simulink model "LQRconlacnguoc"  (R2024b)
settings: Solver=ode45  StartTime=0.0  StopTime=60  FixedStep=0.001  MaxStep=0.01  RelTol=1e-3
values from neighbouring files (symbols this model uses):
  D = [0; 0]    [K_vector_2.m]
libraries: simulink x20, slpidlib x11, slctrl_smc x5, mpclib x1, dspstat3 x1, rllib x1
(part 2 of 3)

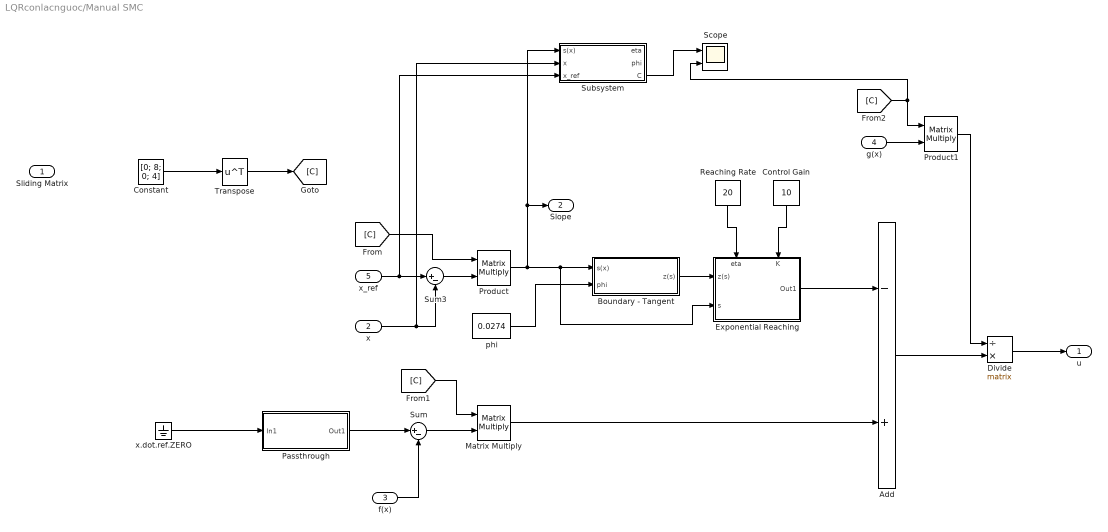
== system LQRconlacnguoc/Manual SMC ==
  Sliding Matrix : Inport
  x : Inport  Port=2
  f(x) : Inport  Port=3
  g(x) : Inport  Port=4
  x_ref : Inport  Port=5
  Add : Sum  Inputs=-+
  Boundary - Tangent : Subsystem
  Constant : Constant  Value=[0; 8; 0; 4]  VectorParams1D=off
  Control Gain : Constant  Value=10
  Divide : Product  Inputs=/*  Multiplication=Matrix(*)
  Exponential Reaching : Subsystem
      settings: PortSchema="{\"entries\":[{\"content\":{\"sides\":[{\"content\":{\"connectorIds\":[\"In1\",\"In2\"]},\"type\":\"ConnectorPlacement.EquallySpacedRectSide\",\"uuid\":\"14532932-ba42-4254-ad37-14ae2c40c086\"},{\"content\":{\"connectorIds\":[\"Out1\"],\"side\":\"RIGHT\"},\"type\":\"ConnectorPlacement.EquallySpacedRectSide\",\"uuid\":\"b67c1209-83dd-4fb0-99c8-05226babf43d\"},{\"content\":{\"connectorIds\":[\"In3\",\"In4\"],\"side\":\"TOP\"},\"type\":\"ConnectorPlacement.EquallySpacedRectSide\",\"uuid\":\"11cfd510-8790-4762-abc8-282610a147ed\"}]},\"type\":\"ConnectorPlacement.EquallySpacedConnector\",\"uuid\":\"c799e45e-6b6c-4526-9867-c33aadee095c\"}],\"packageUris\":[\"http://schema.mathworks.com/mf0/Connector/R2020b\"],\"version\":\"1.0\"}"
  Matrix Multiply : Product  Multiplication=Matrix(*)
  Passthrough : Subsystem  Variant=on
  Product : Product  Multiplication=Matrix(*)
  Product1 : Product  Multiplication=Matrix(*)
  Reaching Rate : Constant  Value=20
  Scope : Scope  NumInputPorts=2
  Subsystem : Subsystem
  Sum : Sum  Inputs=|+-
  Sum3 : Sum  Inputs=|+-
  Transpose : Math  Operator=transpose
  phi : Constant  Value=0.0274
  x.dot.ref.ZERO : Ground
  u : Outport
  Slope : Outport  Port=2
  wires:
  Transpose/1 -> [C]
  [C] -> Product/1
  x/1 -> Subsystem/2(x), Sum3/2
  x_ref/1 -> Subsystem/3(x_ref), Sum3/1
  Sum3/1 -> Product/2
  x.dot.ref.ZERO/1 -> Passthrough/1(In1)
  Passthrough/1(Out1) -> Sum/1
  f(x)/1 -> Sum/2
  Sum/1 -> Matrix Multiply/2
  [C] -> Matrix Multiply/1
  Product/1 -> Subsystem/1(s(x)), Slope/1, Exponential Reaching/2(s), Boundary - Tangent/1(s(x))
  phi/1 -> Boundary - Tangent/2(phi)
  Reaching Rate/1 -> Exponential Reaching/3(eta)
  Control Gain/1 -> Exponential Reaching/4(K)
  Boundary - Tangent/1(z(s)) -> Exponential Reaching/1(z(s))
  Exponential Reaching/1(Out1) -> Add/1
  Matrix Multiply/1 -> Add/2
  [C] -> Scope/2, Product1/1
  g(x)/1 -> Product1/2
  Add/1 -> Divide/2
  Product1/1 -> Divide/1
  Divide/1 -> u/1
  Constant/1 -> Transpose/1
  Subsystem/3(C) -> Scope/1

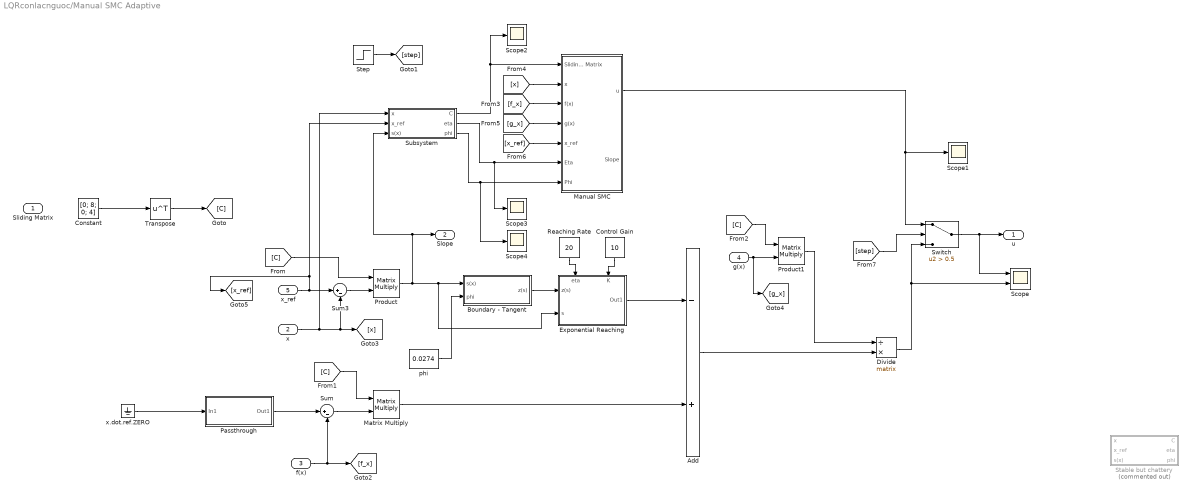
== system LQRconlacnguoc/Manual SMC Adaptive ==
  Sliding Matrix : Inport
  x : Inport  Port=2
  f(x) : Inport  Port=3
  g(x) : Inport  Port=4
  x_ref : Inport  Port=5
  Add : Sum  Inputs=-+
  Boundary - Tangent : Subsystem
  Constant : Constant  Value=[0; 8; 0; 4]  VectorParams1D=off
  Control Gain : Constant  Value=10
  Divide : Product  Inputs=/*  Multiplication=Matrix(*)
  Exponential Reaching : Subsystem
      settings: PortSchema="{\"entries\":[{\"content\":{\"sides\":[{\"content\":{\"connectorIds\":[\"In1\",\"In2\"]},\"type\":\"ConnectorPlacement.EquallySpacedRectSide\",\"uuid\":\"14532932-ba42-4254-ad37-14ae2c40c086\"},{\"content\":{\"connectorIds\":[\"Out1\"],\"side\":\"RIGHT\"},\"type\":\"ConnectorPlacement.EquallySpacedRectSide\",\"uuid\":\"b67c1209-83dd-4fb0-99c8-05226babf43d\"},{\"content\":{\"connectorIds\":[\"In3\",\"In4\"],\"side\":\"TOP\"},\"type\":\"ConnectorPlacement.EquallySpacedRectSide\",\"uuid\":\"11cfd510-8790-4762-abc8-282610a147ed\"}]},\"type\":\"ConnectorPlacement.EquallySpacedConnector\",\"uuid\":\"c799e45e-6b6c-4526-9867-c33aadee095c\"}],\"packageUris\":[\"http://schema.mathworks.com/mf0/Connector/R2020b\"],\"version\":\"1.0\"}"
  Manual SMC : Subsystem
  Matrix Multiply : Product  Multiplication=Matrix(*)
  Passthrough : Subsystem  Variant=on
  Product : Product  Multiplication=Matrix(*)
  Product1 : Product  Multiplication=Matrix(*)
  Reaching Rate : Constant  Value=20
  Scope : Scope  NumInputPorts=2
  Scope{1..4} (4 alike) : Scope
  Stable but chattery : Subsystem  Commented=on
  Step : Step  SampleTime=0.1
  Subsystem : Subsystem
  Sum : Sum  Inputs=|+-
  Sum3 : Sum  Inputs=|+-
  Switch : Switch  Criteria=u2 > Threshold  Threshold=0.5  SaturateOnIntegerOverflow=off  InputSameDT=off
  Transpose : Math  Operator=transpose
  phi : Constant  Value=0.0274
  x.dot.ref.ZERO : Ground
  u : Outport
  Slope : Outport  Port=2
  wires:
  Transpose/1 -> [C]
  [C] -> Product/1
  x/1 -> Subsystem/1(x), [x], Sum3/2
  x_ref/1 -> [x_ref], Subsystem/2(x_ref), Sum3/1
  Sum3/1 -> Product/2
  x.dot.ref.ZERO/1 -> Passthrough/1(In1)
  Passthrough/1(Out1) -> Sum/1
  f(x)/1 -> [f_x], Sum/2
  Sum/1 -> Matrix Multiply/2
  [C] -> Matrix Multiply/1
  Product/1 -> Subsystem/3(s(x)), Slope/1, Exponential Reaching/2(s), Boundary - Tangent/1(s(x))
  Boundary - Tangent/1(z(s)) -> Exponential Reaching/1(z(s))
  Exponential Reaching/1(Out1) -> Add/1
  Matrix Multiply/1 -> Add/2
  [C] -> Product1/1
  g(x)/1 -> [g_x], Product1/2
  Add/1 -> Divide/2
  Product1/1 -> Divide/1
  Control Gain/1 -> Exponential Reaching/4(K)
  Constant/1 -> Transpose/1
  Reaching Rate/1 -> Exponential Reaching/3(eta)
  Step/1 -> [step]
  phi/1 -> Boundary - Tangent/2(phi)
  Subsystem/1(C) -> Manual SMC/1(Sliding Matrix), Scope2/1
  Subsystem/2(eta) -> Manual SMC/6(Eta), Scope3/1
  Subsystem/3(phi) -> Manual SMC/7(Phi), Scope4/1
  [x] -> Manual SMC/2(x)
  [f_x] -> Manual SMC/3(f(x))
  [g_x] -> Manual SMC/4(g(x))
  [x_ref] -> Manual SMC/5(x_ref)
  Divide/1 -> Scope/2, Switch/3
  [step] -> Switch/2
  Manual SMC/1(u) -> Switch/1, Scope1/1
  Switch/1 -> Scope/1, u/1

== system LQRconlacnguoc/PI ==
  Actual Position : Inport
  Reference : Inport  Port=2
  Gain I : Gain  Gain=3.5
  Gain K : Gain  Gain=0
  Integrator : Integrator  LimitOutput=on
  Lowpass : TransferFcn  Denominator=[1 1]
  Scope : Scope
  Sum : Sum  Inputs=|+-
  Sum1 : Sum  Inputs=|++
  Out : Outport
  wires:
  Reference/1 -> Sum/1
  Sum/1 -> Gain I/1, Gain K/1
  Gain I/1 -> Integrator/1
  Gain K/1 -> Sum1/1
  Integrator/1 -> Scope/1, Sum1/2
  Actual Position/1 -> Sum/2
  Sum1/1 -> Lowpass/1
  Lowpass/1 -> Out/1

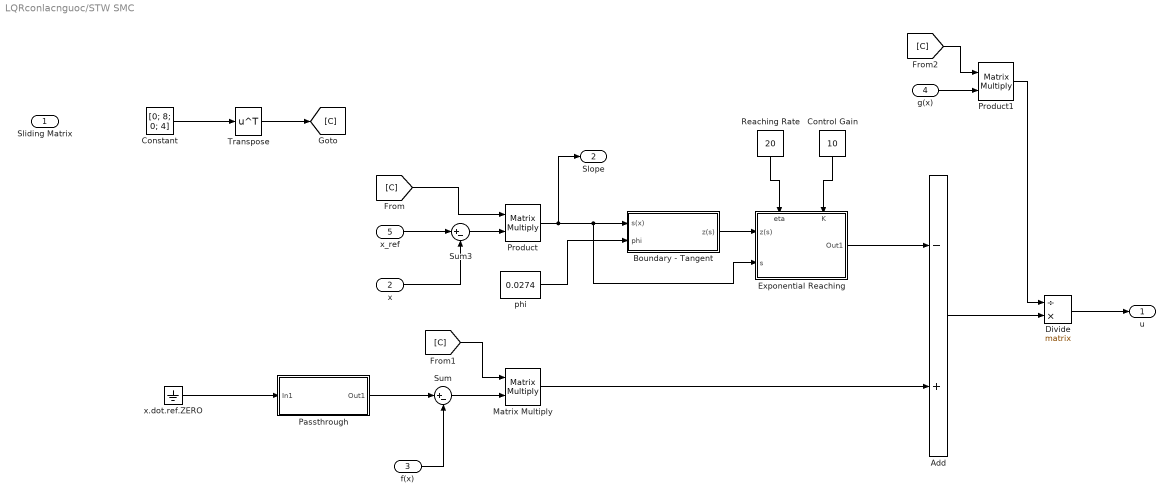
== system LQRconlacnguoc/STW SMC ==
  Sliding Matrix : Inport
  x : Inport  Port=2
  f(x) : Inport  Port=3
  g(x) : Inport  Port=4
  x_ref : Inport  Port=5
  Add : Sum  Inputs=-+
  Boundary - Tangent : Subsystem
  Constant : Constant  Value=[0; 8; 0; 4]  VectorParams1D=off
  Control Gain : Constant  Value=10
  Divide : Product  Inputs=/*  Multiplication=Matrix(*)
  Exponential Reaching : Subsystem
      settings: PortSchema="{\"entries\":[{\"content\":{\"sides\":[{\"content\":{\"connectorIds\":[\"In1\",\"In2\"]},\"type\":\"ConnectorPlacement.EquallySpacedRectSide\",\"uuid\":\"14532932-ba42-4254-ad37-14ae2c40c086\"},{\"content\":{\"connectorIds\":[\"Out1\"],\"side\":\"RIGHT\"},\"type\":\"ConnectorPlacement.EquallySpacedRectSide\",\"uuid\":\"b67c1209-83dd-4fb0-99c8-05226babf43d\"},{\"content\":{\"connectorIds\":[\"In3\",\"In4\"],\"side\":\"TOP\"},\"type\":\"ConnectorPlacement.EquallySpacedRectSide\",\"uuid\":\"11cfd510-8790-4762-abc8-282610a147ed\"}]},\"type\":\"ConnectorPlacement.EquallySpacedConnector\",\"uuid\":\"c799e45e-6b6c-4526-9867-c33aadee095c\"}],\"packageUris\":[\"http://schema.mathworks.com/mf0/Connector/R2020b\"],\"version\":\"1.0\"}"
  Matrix Multiply : Product  Multiplication=Matrix(*)
  Passthrough : Subsystem  Variant=on
  Product : Product  Multiplication=Matrix(*)
  Product1 : Product  Multiplication=Matrix(*)
  Reaching Rate : Constant  Value=20
  Sum : Sum  Inputs=|+-
  Sum3 : Sum  Inputs=|+-
  Transpose : Math  Operator=transpose
  phi : Constant  Value=0.0274
  x.dot.ref.ZERO : Ground
  u : Outport
  Slope : Outport  Port=2
  wires:
  Transpose/1 -> [C]
  [C] -> Product/1
  x/1 -> Sum3/2
  x_ref/1 -> Sum3/1
  Sum3/1 -> Product/2
  x.dot.ref.ZERO/1 -> Passthrough/1(In1)
  Passthrough/1(Out1) -> Sum/1
  f(x)/1 -> Sum/2
  Sum/1 -> Matrix Multiply/2
  [C] -> Matrix Multiply/1
  Product/1 -> Slope/1, Exponential Reaching/2(s), Boundary - Tangent/1(s(x))
  phi/1 -> Boundary - Tangent/2(phi)
  Reaching Rate/1 -> Exponential Reaching/3(eta)
  Control Gain/1 -> Exponential Reaching/4(K)
  Boundary - Tangent/1(z(s)) -> Exponential Reaching/1(z(s))
  Exponential Reaching/1(Out1) -> Add/1
  Matrix Multiply/1 -> Add/2
  [C] -> Product1/1
  g(x)/1 -> Product1/2
  Add/1 -> Divide/2
  Product1/1 -> Divide/1
  Divide/1 -> u/1
  Constant/1 -> Transpose/1

== system LQRconlacnguoc/Subsystem ==
  x_ref : Inport
  x1 : Inport  Port=2
  x2 : Inport  Port=3
  v1 : Inport  Port=4
  v2 : Inport  Port=5
  MATLAB Function : MATLAB Function  TreatAsAtomicUnit=on  SystemSampleTime=0.01
  MATLAB Function1 : MATLAB Function  TreatAsAtomicUnit=on  SystemSampleTime=0.01
  MATLAB Function2 : MATLAB Function  TreatAsAtomicUnit=on  SystemSampleTime=0.01
  k_P : Outport
  k_I : Outport  Port=2
  k_D : Outport  Port=3
  wires:
  x1/1 -> MATLAB Function1/1(x1), MATLAB Function2/1(x1), MATLAB Function/1(x1)
  x2/1 -> MATLAB Function2/2(x2), MATLAB Function1/2(x2), MATLAB Function/2(x2)
  v1/1 -> MATLAB Function1/3(v1), MATLAB Function2/3(v1), MATLAB Function/3(v1)
  v2/1 -> MATLAB Function2/4(v2), MATLAB Function1/4(v2), MATLAB Function/4(v2)
  MATLAB Function2/1(Ki_out) -> k_I/1
  MATLAB Function/1(Kp_out) -> k_P/1
  MATLAB Function1/1(Kd_out) -> k_D/1
  x_ref/1 -> MATLAB Function2/5(x2_ref), MATLAB Function1/5(x2_ref), MATLAB Function/5(x2_ref)

== system LQRconlacnguoc/Subsystem1 ==
  u : Inport
  Mux1 : Mux  Inputs=3
  Mux2 : Mux  Inputs=3
  thetadot : Integrator
  thetadotdot : Fcn  Expr=(u(1)*cos(u(2)) -(2.4+0.23)*9.8*sin(u(2))+0.23*0.36*cos(u(2))*sin(u(2))*(u(3))^2)/ (0.23*0.36*(cos(u(2)))^2 - (2.4+0.23)*0.36)
  thetha : Integrator
  x : Integrator
  xdot : Integrator
  xdotdot : Fcn  Expr="(u(1) + 0.23*0.36*sin(u(2))*(u(3))^2  - 0.23*9.8*cos(u(2))*sin(u(2))) / (2.4 + 0.23 - 0.23*(cos(u(2)))^2)"
  góc : Outport
  góc dot : Outport  Port=2
  vị trí : Outport  Port=3
  vị trí dot : Outport  Port=4
  wires:
  u/1 -> Mux2/1, Mux1/1
  Mux1/1 -> xdotdot/1
  thetadotdot/1 -> thetadot/1
  thetadot/1 -> góc dot/1, thetha/1, Mux2/3, Mux1/3
  Mux2/1 -> thetadotdot/1
  thetha/1 -> Mux1/2, Mux2/2, góc/1
  xdotdot/1 -> xdot/1
  xdot/1 -> x/1, vị trí dot/1
  x/1 -> vị trí/1

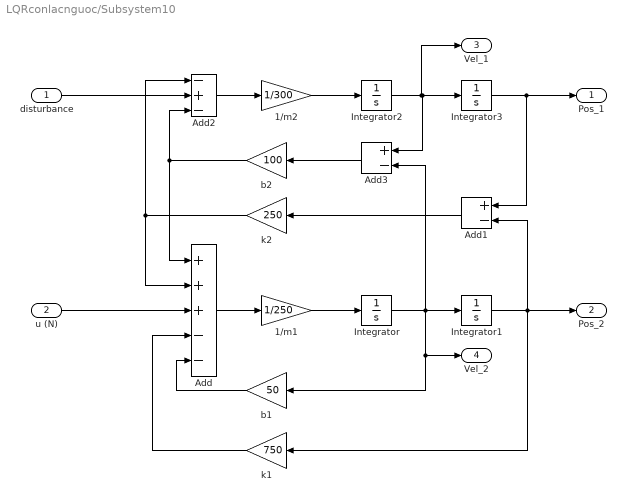
== system LQRconlacnguoc/Subsystem10 ==
  disturbance : Inport
  u (N) : Inport  Port=2
  1/m1 : Gain  Gain=1/250
  1/m2 : Gain  Gain=1/300
  Add : Sum  Inputs=+++--
  Add1 : Sum  Inputs=+-
  Add2 : Sum  Inputs=-+-
  Add3 : Sum  Inputs=+-
  Integrator{,1..3} (4 alike) : Integrator
  b1 : Gain  Gain=50
  b2 : Gain  Gain=100
  k1 : Gain  Gain=750
  k2 : Gain  Gain=250
  Pos_1 : Outport
  Pos_2 : Outport  Port=2
  Vel_1 : Outport  Port=3
  Vel_2 : Outport  Port=4
  wires:
  Add/1 -> 1/m1/1
  1/m1/1 -> Integrator/1
  Integrator/1 -> Add3/2, Integrator1/1, b1/1, Vel_2/1
  Integrator1/1 -> k1/1, Pos_2/1, Add1/2
  Add2/1 -> 1/m2/1
  1/m2/1 -> Integrator2/1
  Integrator2/1 -> Vel_1/1, Add3/1, Integrator3/1
  Add3/1 -> b2/1
  b2/1 -> Add2/3, Add/1
  Add1/1 -> k2/1
  Integrator3/1 -> Pos_1/1, Add1/1
  u (N)/1 -> Add/3
  b1/1 -> Add/5
  k1/1 -> Add/4
  k2/1 -> Add2/1, Add/2
  disturbance/1 -> Add2/2

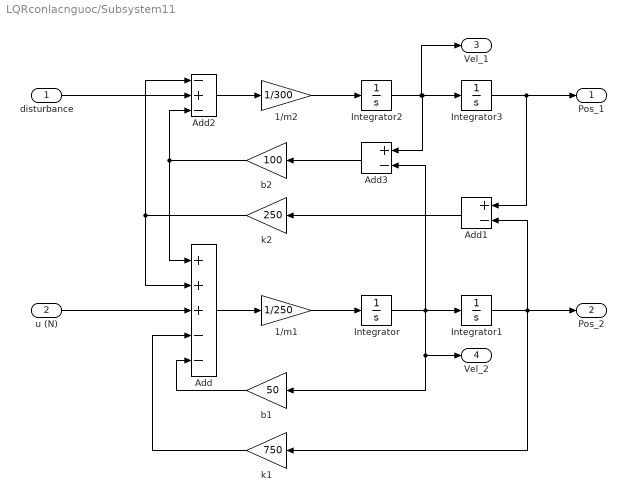
== system LQRconlacnguoc/Subsystem11 ==
  disturbance : Inport
  u (N) : Inport  Port=2
  1/m1 : Gain  Gain=1/250
  1/m2 : Gain  Gain=1/300
  Add : Sum  Inputs=+++--
  Add1 : Sum  Inputs=+-
  Add2 : Sum  Inputs=-+-
  Add3 : Sum  Inputs=+-
  Integrator{,1..3} (4 alike) : Integrator
  b1 : Gain  Gain=50
  b2 : Gain  Gain=100
  k1 : Gain  Gain=750
  k2 : Gain  Gain=250
  Pos_1 : Outport
  Pos_2 : Outport  Port=2
  Vel_1 : Outport  Port=3
  Vel_2 : Outport  Port=4
  wires:
  Add/1 -> 1/m1/1
  1/m1/1 -> Integrator/1
  Integrator/1 -> Add3/2, Integrator1/1, b1/1, Vel_2/1
  Integrator1/1 -> k1/1, Pos_2/1, Add1/2
  Add2/1 -> 1/m2/1
  1/m2/1 -> Integrator2/1
  Integrator2/1 -> Vel_1/1, Add3/1, Integrator3/1
  Add3/1 -> b2/1
  b2/1 -> Add2/3, Add/1
  Add1/1 -> k2/1
  Integrator3/1 -> Pos_1/1, Add1/1
  u (N)/1 -> Add/3
  b1/1 -> Add/5
  k1/1 -> Add/4
  k2/1 -> Add2/1, Add/2
  disturbance/1 -> Add2/2

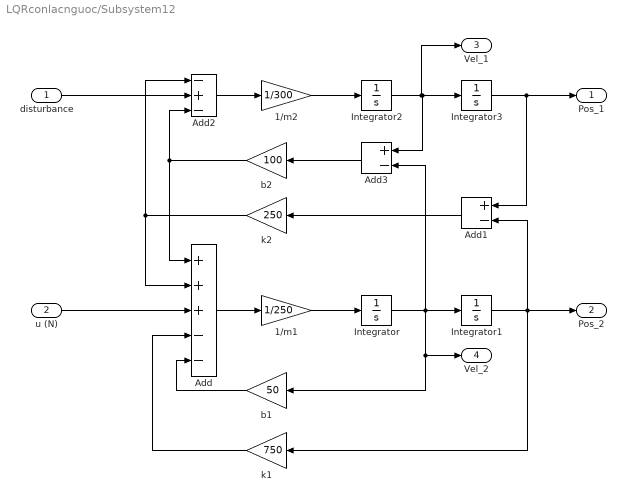
== system LQRconlacnguoc/Subsystem12 ==
  disturbance : Inport
  u (N) : Inport  Port=2
  1/m1 : Gain  Gain=1/250
  1/m2 : Gain  Gain=1/300
  Add : Sum  Inputs=+++--
  Add1 : Sum  Inputs=+-
  Add2 : Sum  Inputs=-+-
  Add3 : Sum  Inputs=+-
  Integrator{,1..3} (4 alike) : Integrator
  b1 : Gain  Gain=50
  b2 : Gain  Gain=100
  k1 : Gain  Gain=750
  k2 : Gain  Gain=250
  Pos_1 : Outport
  Pos_2 : Outport  Port=2
  Vel_1 : Outport  Port=3
  Vel_2 : Outport  Port=4
  wires:
  Add/1 -> 1/m1/1
  1/m1/1 -> Integrator/1
  Integrator/1 -> Add3/2, Integrator1/1, b1/1, Vel_2/1
  Integrator1/1 -> k1/1, Pos_2/1, Add1/2
  Add2/1 -> 1/m2/1
  1/m2/1 -> Integrator2/1
  Integrator2/1 -> Vel_1/1, Add3/1, Integrator3/1
  Add3/1 -> b2/1
  b2/1 -> Add2/3, Add/1
  Add1/1 -> k2/1
  Integrator3/1 -> Pos_1/1, Add1/1
  u (N)/1 -> Add/3
  b1/1 -> Add/5
  k1/1 -> Add/4
  k2/1 -> Add2/1, Add/2
  disturbance/1 -> Add2/2

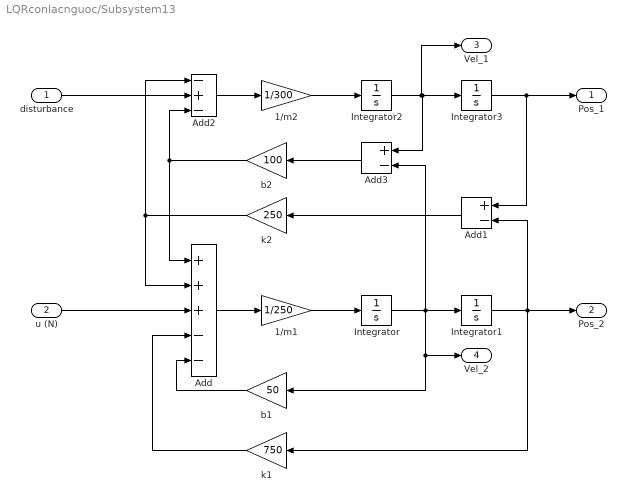
== system LQRconlacnguoc/Subsystem13 ==
  disturbance : Inport
  u (N) : Inport  Port=2
  1/m1 : Gain  Gain=1/250
  1/m2 : Gain  Gain=1/300
  Add : Sum  Inputs=+++--
  Add1 : Sum  Inputs=+-
  Add2 : Sum  Inputs=-+-
  Add3 : Sum  Inputs=+-
  Integrator{,1..3} (4 alike) : Integrator
  b1 : Gain  Gain=50
  b2 : Gain  Gain=100
  k1 : Gain  Gain=750
  k2 : Gain  Gain=250
  Pos_1 : Outport
  Pos_2 : Outport  Port=2
  Vel_1 : Outport  Port=3
  Vel_2 : Outport  Port=4
  wires:
  Add/1 -> 1/m1/1
  1/m1/1 -> Integrator/1
  Integrator/1 -> Add3/2, Integrator1/1, b1/1, Vel_2/1
  Integrator1/1 -> k1/1, Pos_2/1, Add1/2
  Add2/1 -> 1/m2/1
  1/m2/1 -> Integrator2/1
  Integrator2/1 -> Vel_1/1, Add3/1, Integrator3/1
  Add3/1 -> b2/1
  b2/1 -> Add2/3, Add/1
  Add1/1 -> k2/1
  Integrator3/1 -> Pos_1/1, Add1/1
  u (N)/1 -> Add/3
  b1/1 -> Add/5
  k1/1 -> Add/4
  k2/1 -> Add2/1, Add/2
  disturbance/1 -> Add2/2

== system LQRconlacnguoc/Subsystem14 ==
  u : Inport
  Mux1 : Mux  Inputs=3
  Mux2 : Mux  Inputs=3
  thetadot : Integrator
  thetadotdot : Fcn  Expr=(u(1)*cos(u(2)) -(2.4+0.23)*9.8*sin(u(2))+0.23*0.36*cos(u(2))*sin(u(2))*(u(3))^2)/ (0.23*0.36*(cos(u(2)))^2 - (2.4+0.23)*0.36)
  thetha : Integrator
  x : Integrator
  xdot : Integrator
  xdotdot : Fcn  Expr="(u(1) + 0.23*0.36*sin(u(2))*(u(3))^2  - 0.23*9.8*cos(u(2))*sin(u(2))) / (2.4 + 0.23 - 0.23*(cos(u(2)))^2)"
  theta : Outport
  theta_dot : Outport  Port=2
  pos : Outport  Port=3
  pos_dot : Outport  Port=4
  wires:
  u/1 -> Mux2/1, Mux1/1
  Mux1/1 -> xdotdot/1
  thetadotdot/1 -> thetadot/1
  thetadot/1 -> Mux1/3, Mux2/3, thetha/1, theta_dot/1
  Mux2/1 -> thetadotdot/1
  thetha/1 -> Mux1/2, Mux2/2, theta/1
  xdotdot/1 -> xdot/1
  xdot/1 -> x/1, pos_dot/1
  x/1 -> pos/1

== system LQRconlacnguoc/Subsystem15 ==
  u : Inport
  Mux1 : Mux  Inputs=3
  Mux2 : Mux  Inputs=3
  thetadot : Integrator
  thetadotdot : Fcn  Expr=(u(1)*cos(u(2)) -(2.4+0.23)*9.8*sin(u(2))+0.23*0.36*cos(u(2))*sin(u(2))*(u(3))^2)/ (0.23*0.36*(cos(u(2)))^2 - (2.4+0.23)*0.36)
  thetha : Integrator
  x : Integrator
  xdot : Integrator
  xdotdot : Fcn  Expr="(u(1) + 0.23*0.36*sin(u(2))*(u(3))^2  - 0.23*9.8*cos(u(2))*sin(u(2))) / (2.4 + 0.23 - 0.23*(cos(u(2)))^2)"
  theta : Outport
  theta_dot : Outport  Port=2
  pos : Outport  Port=3
  pos_dot : Outport  Port=4
  wires:
  u/1 -> Mux2/1, Mux1/1
  Mux1/1 -> xdotdot/1
  thetadotdot/1 -> thetadot/1
  thetadot/1 -> Mux1/3, Mux2/3, thetha/1, theta_dot/1
  Mux2/1 -> thetadotdot/1
  thetha/1 -> Mux1/2, Mux2/2, theta/1
  xdotdot/1 -> xdot/1
  xdot/1 -> x/1, pos_dot/1
  x/1 -> pos/1

== system LQRconlacnguoc/Subsystem16 ==
  u : Inport
  Mux1 : Mux  Inputs=3
  Mux2 : Mux  Inputs=3
  theta'' : Fcn  Expr=(u(1)*cos(u(2)) -(2.4+0.23)*9.8*sin(u(2))+0.23*0.36*cos(u(2))*sin(u(2))*(u(3))^2)/ (0.23*0.36*(cos(u(2)))^2 - (2.4+0.23)*0.36)
  thetadot : Integrator
  thetha : Integrator
  x : Integrator
  x'' : Fcn  Expr="(u(1) + 0.23*0.36*sin(u(2))*(u(3))^2  - 0.23*9.8*cos(u(2))*sin(u(2))) / (2.4 + 0.23 - 0.23*(cos(u(2)))^2)"
  xdot : Integrator
  theta : Outport
  theta_dot : Outport  Port=2
  pos : Outport  Port=3
  pos_dot : Outport  Port=4
  wires:
  u/1 -> Mux2/1, Mux1/1
  Mux1/1 -> x''/1
  theta''/1 -> thetadot/1
  thetadot/1 -> Mux1/3, Mux2/3, thetha/1, theta_dot/1
  Mux2/1 -> theta''/1
  thetha/1 -> Mux1/2, Mux2/2, theta/1
  x''/1 -> xdot/1
  xdot/1 -> x/1, pos_dot/1
  x/1 -> pos/1

== system LQRconlacnguoc/Subsystem2 ==
  u : Inport
  Mux1 : Mux  Inputs=3
  Mux2 : Mux  Inputs=3
  thetadot : Integrator
  thetadotdot : Fcn  Expr=(u(1)*cos(u(2)) -(2.4+0.23)*9.8*sin(u(2))+0.23*0.36*cos(u(2))*sin(u(2))*(u(3))^2)/ (0.23*0.36*(cos(u(2)))^2 - (2.4+0.23)*0.36)
  thetha : Integrator
  x : Integrator
  xdot : Integrator
  xdotdot : Fcn  Expr="(u(1) + 0.23*0.36*sin(u(2))*(u(3))^2  - 0.23*9.8*cos(u(2))*sin(u(2))) / (2.4 + 0.23 - 0.23*(cos(u(2)))^2)"
  góc : Outport
  góc dot : Outport  Port=2
  vị trí : Outport  Port=3
  vị trí dot : Outport  Port=4
  wires:
  u/1 -> Mux2/1, Mux1/1
  Mux1/1 -> xdotdot/1
  thetadotdot/1 -> thetadot/1
  thetadot/1 -> góc dot/1, thetha/1, Mux2/3, Mux1/3
  Mux2/1 -> thetadotdot/1
  thetha/1 -> Mux1/2, Mux2/2, góc/1
  xdotdot/1 -> xdot/1
  xdot/1 -> x/1, vị trí dot/1
  x/1 -> vị trí/1

== system LQRconlacnguoc/Subsystem3 ==
  u : Inport
  Mux1 : Mux  Inputs=3
  Mux2 : Mux  Inputs=3
  thetadot : Integrator
  thetadotdot : Fcn  Expr=(u(1)*cos(u(2)) -(2.4+0.23)*9.8*sin(u(2))+0.23*0.36*cos(u(2))*sin(u(2))*(u(3))^2)/ (0.23*0.36*(cos(u(2)))^2 - (2.4+0.23)*0.36)
  thetha : Integrator
  x : Integrator
  xdot : Integrator
  xdotdot : Fcn  Expr="(u(1) + 0.23*0.36*sin(u(2))*(u(3))^2  - 0.23*9.8*cos(u(2))*sin(u(2))) / (2.4 + 0.23 - 0.23*(cos(u(2)))^2)"
  góc : Outport
  góc dot : Outport  Port=2
  vị trí : Outport  Port=3
  vị trí dot : Outport  Port=4
  wires:
  u/1 -> Mux2/1, Mux1/1
  Mux1/1 -> xdotdot/1
  thetadotdot/1 -> thetadot/1
  thetadot/1 -> Mux1/3, Mux2/3, thetha/1, góc dot/1
  Mux2/1 -> thetadotdot/1
  thetha/1 -> Mux1/2, Mux2/2, góc/1
  xdotdot/1 -> xdot/1
  xdot/1 -> x/1, vị trí dot/1
  x/1 -> vị trí/1

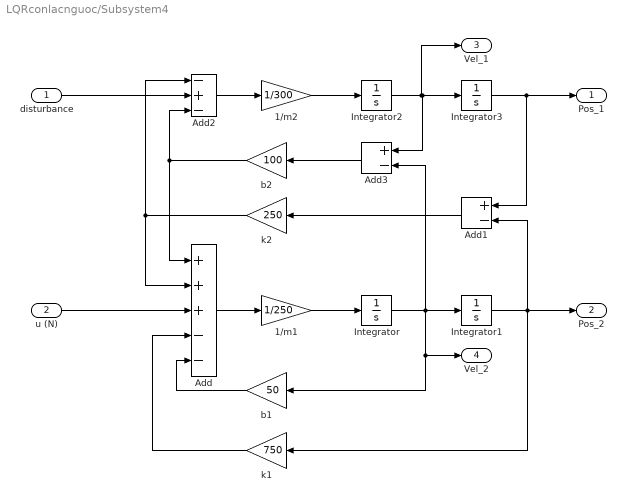
== system LQRconlacnguoc/Subsystem4 ==
  disturbance : Inport
  u (N) : Inport  Port=2
  1/m1 : Gain  Gain=1/250
  1/m2 : Gain  Gain=1/300
  Add : Sum  Inputs=+++--
  Add1 : Sum  Inputs=+-
  Add2 : Sum  Inputs=-+-
  Add3 : Sum  Inputs=+-
  Integrator{,1..3} (4 alike) : Integrator
  b1 : Gain  Gain=50
  b2 : Gain  Gain=100
  k1 : Gain  Gain=750
  k2 : Gain  Gain=250
  Pos_1 : Outport
  Pos_2 : Outport  Port=2
  Vel_1 : Outport  Port=3
  Vel_2 : Outport  Port=4
  wires:
  Add/1 -> 1/m1/1
  1/m1/1 -> Integrator/1
  Integrator/1 -> Add3/2, Integrator1/1, b1/1, Vel_2/1
  Integrator1/1 -> k1/1, Pos_2/1, Add1/2
  Add2/1 -> 1/m2/1
  1/m2/1 -> Integrator2/1
  Integrator2/1 -> Vel_1/1, Add3/1, Integrator3/1
  Add3/1 -> b2/1
  b2/1 -> Add2/3, Add/1
  Add1/1 -> k2/1
  Integrator3/1 -> Pos_1/1, Add1/1
  u (N)/1 -> Add/3
  b1/1 -> Add/5
  k1/1 -> Add/4
  k2/1 -> Add2/1, Add/2
  disturbance/1 -> Add2/2

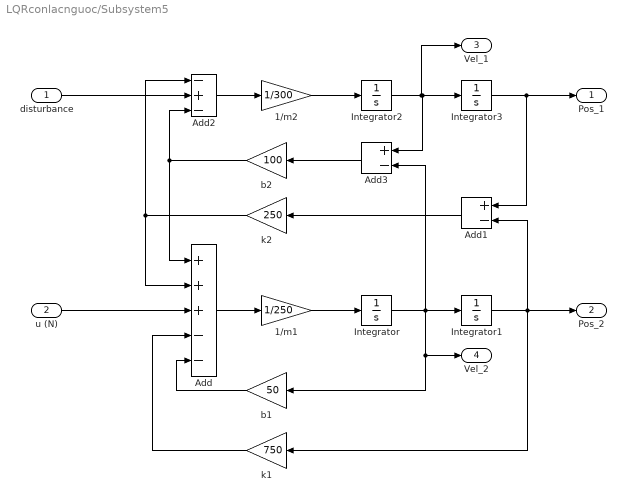
== system LQRconlacnguoc/Subsystem5 ==
  disturbance : Inport
  u (N) : Inport  Port=2
  1/m1 : Gain  Gain=1/250
  1/m2 : Gain  Gain=1/300
  Add : Sum  Inputs=+++--
  Add1 : Sum  Inputs=+-
  Add2 : Sum  Inputs=-+-
  Add3 : Sum  Inputs=+-
  Integrator{,1..3} (4 alike) : Integrator
  b1 : Gain  Gain=50
  b2 : Gain  Gain=100
  k1 : Gain  Gain=750
  k2 : Gain  Gain=250
  Pos_1 : Outport
  Pos_2 : Outport  Port=2
  Vel_1 : Outport  Port=3
  Vel_2 : Outport  Port=4
  wires:
  Add/1 -> 1/m1/1
  1/m1/1 -> Integrator/1
  Integrator/1 -> Add3/2, Integrator1/1, b1/1, Vel_2/1
  Integrator1/1 -> k1/1, Pos_2/1, Add1/2
  Add2/1 -> 1/m2/1
  1/m2/1 -> Integrator2/1
  Integrator2/1 -> Vel_1/1, Add3/1, Integrator3/1
  Add3/1 -> b2/1
  b2/1 -> Add2/3, Add/1
  Add1/1 -> k2/1
  Integrator3/1 -> Pos_1/1, Add1/1
  u (N)/1 -> Add/3
  b1/1 -> Add/5
  k1/1 -> Add/4
  k2/1 -> Add2/1, Add/2
  disturbance/1 -> Add2/2

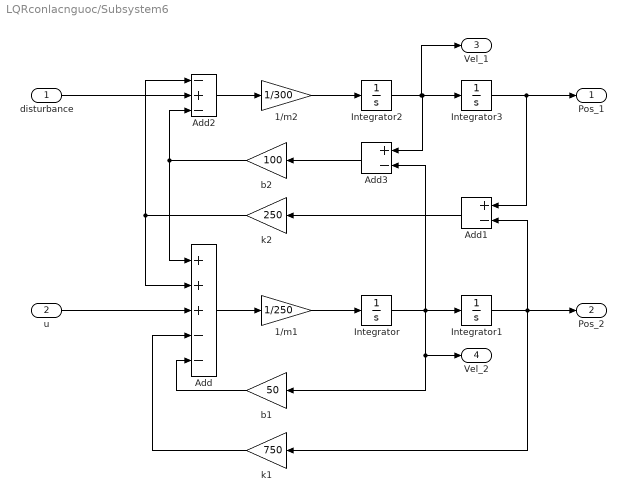
== system LQRconlacnguoc/Subsystem6 ==
  disturbance : Inport
  u : Inport  Port=2
  1/m1 : Gain  Gain=1/250
  1/m2 : Gain  Gain=1/300
  Add : Sum  Inputs=+++--
  Add1 : Sum  Inputs=+-
  Add2 : Sum  Inputs=-+-
  Add3 : Sum  Inputs=+-
  Integrator{,1..3} (4 alike) : Integrator
  b1 : Gain  Gain=50
  b2 : Gain  Gain=100
  k1 : Gain  Gain=750
  k2 : Gain  Gain=250
  Pos_1 : Outport
  Pos_2 : Outport  Port=2
  Vel_1 : Outport  Port=3
  Vel_2 : Outport  Port=4
  wires:
  Add/1 -> 1/m1/1
  1/m1/1 -> Integrator/1
  Integrator/1 -> Add3/2, Integrator1/1, b1/1, Vel_2/1
  Integrator1/1 -> k1/1, Pos_2/1, Add1/2
  Add2/1 -> 1/m2/1
  1/m2/1 -> Integrator2/1
  Integrator2/1 -> Vel_1/1, Add3/1, Integrator3/1
  Add3/1 -> b2/1
  b2/1 -> Add2/3, Add/1
  Add1/1 -> k2/1
  Integrator3/1 -> Pos_1/1, Add1/1
  u/1 -> Add/3
  b1/1 -> Add/5
  k1/1 -> Add/4
  k2/1 -> Add2/1, Add/2
  disturbance/1 -> Add2/2

== system LQRconlacnguoc/Subsystem7 ==
  disturbance : Inport
  u (N) : Inport  Port=2
  1/m1 : Gain  Gain=1/250
  1/m2 : Gain  Gain=1/300
  Add : Sum  Inputs=+++--
  Add1 : Sum  Inputs=+-
  Add2 : Sum  Inputs=-+-
  Add3 : Sum  Inputs=+-
  Integrator{,1..3} (4 alike) : Integrator
  b1 : Gain  Gain=50
  b2 : Gain  Gain=100
  k1 : Gain  Gain=750
  k2 : Gain  Gain=250
  Pos_1 : Outport
  Pos_2 : Outport  Port=2
  Vel_1 : Outport  Port=3
  Vel_2 : Outport  Port=4
  wires:
  Add/1 -> 1/m1/1
  1/m1/1 -> Integrator/1
  Integrator/1 -> Add3/2, Integrator1/1, b1/1, Vel_2/1
  Integrator1/1 -> k1/1, Pos_2/1, Add1/2
  Add2/1 -> 1/m2/1
  1/m2/1 -> Integrator2/1
  Integrator2/1 -> Vel_1/1, Add3/1, Integrator3/1
  Add3/1 -> b2/1
  b2/1 -> Add2/3, Add/1
  Add1/1 -> k2/1
  Integrator3/1 -> Pos_1/1, Add1/1
  u (N)/1 -> Add/3
  b1/1 -> Add/5
  k1/1 -> Add/4
  k2/1 -> Add2/1, Add/2
  disturbance/1 -> Add2/2

== system LQRconlacnguoc/Subsystem8 ==
  disturbance : Inport
  u (N) : Inport  Port=2
  1/m1 : Gain  Gain=1/250
  1/m2 : Gain  Gain=1/300
  Add : Sum  Inputs=+++--
  Add1 : Sum  Inputs=+-
  Add2 : Sum  Inputs=-+-
  Add3 : Sum  Inputs=+-
  Integrator{,1..3} (4 alike) : Integrator
  b1 : Gain  Gain=50
  b2 : Gain  Gain=100
  k1 : Gain  Gain=750
  k2 : Gain  Gain=250
  Pos_1 : Outport
  Pos_2 : Outport  Port=2
  Vel_1 : Outport  Port=3
  Vel_2 : Outport  Port=4
  wires:
  Add/1 -> 1/m1/1
  1/m1/1 -> Integrator/1
  Integrator/1 -> Add3/2, Integrator1/1, b1/1, Vel_2/1
  Integrator1/1 -> k1/1, Pos_2/1, Add1/2
  Add2/1 -> 1/m2/1
  1/m2/1 -> Integrator2/1
  Integrator2/1 -> Vel_1/1, Add3/1, Integrator3/1
  Add3/1 -> b2/1
  b2/1 -> Add2/3, Add/1
  Add1/1 -> k2/1
  Integrator3/1 -> Pos_1/1, Add1/1
  u (N)/1 -> Add/3
  b1/1 -> Add/5
  k1/1 -> Add/4
  k2/1 -> Add2/1, Add/2
  disturbance/1 -> Add2/2

== system LQRconlacnguoc/Subsystem9 ==
  disturbance : Inport
  u : Inport  Port=2
  1/m : Gain  Gain=1/250
  Add : Sum  Inputs=++--
  Integrator : Integrator
  Integrator1 : Integrator
  b : Gain  Gain=50
  k : Gain  Gain=750
  x : Outport
  v : Outport  Port=2
  wires:
  Add/1 -> 1/m/1
  1/m/1 -> Integrator/1
  Integrator/1 -> v/1, b/1, Integrator1/1
  Integrator1/1 -> x/1, k/1
  u/1 -> Add/1
  b/1 -> Add/4
  k/1 -> Add/3
  disturbance/1 -> Add/2

== system LQRconlacnguoc/Manual SMC/Boundary - Tangent ==
  s(x) : Inport
  phi : Inport  Port=2
  Divide : Product  Inputs=*/
  Reshape1 : Reshape  OutputDimensionality=Column vector (2-D)
  Reshape2 : Reshape  OutputDimensionality=Column vector (2-D)
  Tanh : Trigonometry  Operator=tanh
  z(s) : Outport
  wires:
  Reshape1/1 -> Divide/2
  Divide/1 -> Tanh/1
  phi/1 -> Reshape1/1
  Reshape2/1 -> Divide/1
  Tanh/1 -> z(s)/1
  s(x)/1 -> Reshape2/1

== system LQRconlacnguoc/Manual SMC/Exponential Reaching ==
  z(s) : Inport
  s : Inport  Port=2
  eta : Inport  Port=3
  K : Inport  Port=4
  Product : Product  Inputs=**
  Product1 : Product
  Sum : Sum  Inputs=--
  Out1 : Outport
  wires:
  z(s)/1 -> Product/2
  eta/1 -> Product/1
  s/1 -> Product1/1
  K/1 -> Product1/2
  Product/1 -> Sum/1
  Product1/1 -> Sum/2
  Sum/1 -> Out1/1

== system LQRconlacnguoc/Manual SMC/Passthrough ==
  note: 1) Add Subsystem or Model blocks as valid variant choices.
      | 2) You cannot connect blocks at this level. At simulation, connectivity is automatically
      | determined, based on the active variant and port name matching.
  In1 : Inport
  Subsystem : Subsystem  VariantControl=true
  Subsystem1 : Subsystem  VariantControl=false
  Out1 : Outport

== system LQRconlacnguoc/Manual SMC/Subsystem ==
  s(x) : Inport
  x : Inport  Port=2
  x_ref : Inport  Port=3
  MATLAB Function : MATLAB Function  TreatAsAtomicUnit=on
  eta : Outport
  phi : Outport  Port=2
  C : Outport  Port=3
  wires:
  s(x)/1 -> MATLAB Function/1(s)
  MATLAB Function/1(eta) -> eta/1
  MATLAB Function/2(phi) -> phi/1
  MATLAB Function/3(C) -> C/1
  x/1 -> MATLAB Function/2(x)
  x_ref/1 -> MATLAB Function/3(x_ref)

== system LQRconlacnguoc/Manual SMC Adaptive/Boundary - Tangent ==
  s(x) : Inport
  phi : Inport  Port=2
  Divide : Product  Inputs=*/
  Reshape1 : Reshape  OutputDimensionality=Column vector (2-D)
  Reshape2 : Reshape  OutputDimensionality=Column vector (2-D)
  Tanh : Trigonometry  Operator=tanh
  z(s) : Outport
  wires:
  Reshape1/1 -> Divide/2
  Divide/1 -> Tanh/1
  phi/1 -> Reshape1/1
  Reshape2/1 -> Divide/1
  Tanh/1 -> z(s)/1
  s(x)/1 -> Reshape2/1

== system LQRconlacnguoc/Manual SMC Adaptive/Exponential Reaching ==
  z(s) : Inport
  s : Inport  Port=2
  eta : Inport  Port=3
  K : Inport  Port=4
  Product : Product  Inputs=**
  Product1 : Product
  Sum : Sum  Inputs=--
  Out1 : Outport
  wires:
  z(s)/1 -> Product/2
  eta/1 -> Product/1
  s/1 -> Product1/1
  K/1 -> Product1/2
  Product/1 -> Sum/1
  Product1/1 -> Sum/2
  Sum/1 -> Out1/1

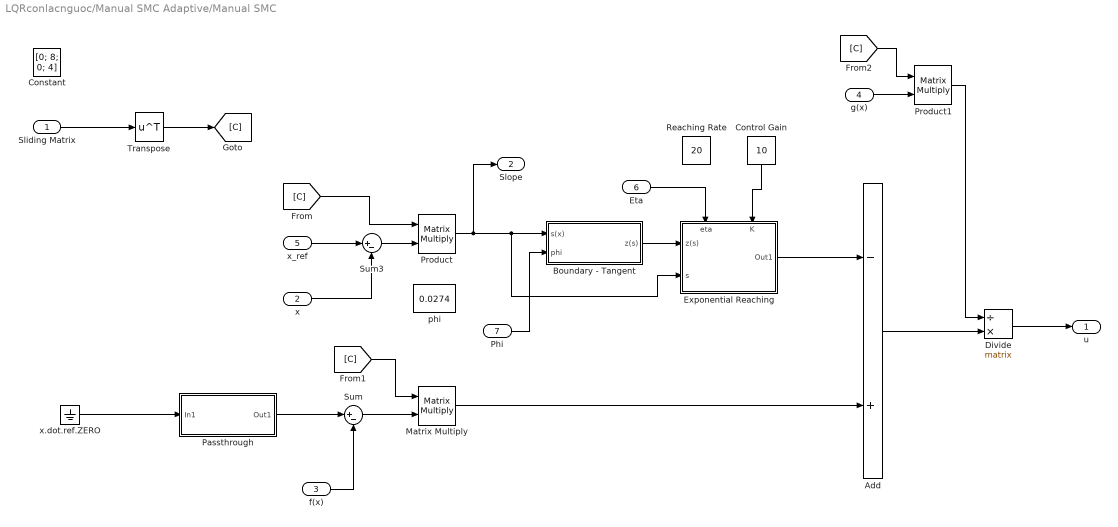
== system LQRconlacnguoc/Manual SMC Adaptive/Manual SMC ==
  Sliding Matrix : Inport
  x : Inport  Port=2
  f(x) : Inport  Port=3
  g(x) : Inport  Port=4
  x_ref : Inport  Port=5
  Eta : Inport  Port=6
  Phi : Inport  Port=7
  Add : Sum  Inputs=-+
  Boundary - Tangent : Subsystem
  Constant : Constant  Value=[0; 8; 0; 4]  VectorParams1D=off
  Control Gain : Constant  Value=10
  Divide : Product  Inputs=/*  Multiplication=Matrix(*)
  Exponential Reaching : Subsystem
      settings: PortSchema="{\"entries\":[{\"content\":{\"sides\":[{\"content\":{\"connectorIds\":[\"In1\",\"In2\"]},\"type\":\"ConnectorPlacement.EquallySpacedRectSide\",\"uuid\":\"14532932-ba42-4254-ad37-14ae2c40c086\"},{\"content\":{\"connectorIds\":[\"Out1\"],\"side\":\"RIGHT\"},\"type\":\"ConnectorPlacement.EquallySpacedRectSide\",\"uuid\":\"b67c1209-83dd-4fb0-99c8-05226babf43d\"},{\"content\":{\"connectorIds\":[\"In3\",\"In4\"],\"side\":\"TOP\"},\"type\":\"ConnectorPlacement.EquallySpacedRectSide\",\"uuid\":\"11cfd510-8790-4762-abc8-282610a147ed\"}]},\"type\":\"ConnectorPlacement.EquallySpacedConnector\",\"uuid\":\"c799e45e-6b6c-4526-9867-c33aadee095c\"}],\"packageUris\":[\"http://schema.mathworks.com/mf0/Connector/R2020b\"],\"version\":\"1.0\"}"
  Matrix Multiply : Product  Multiplication=Matrix(*)
  Passthrough : Subsystem  Variant=on
  Product : Product  Multiplication=Matrix(*)
  Product1 : Product  Multiplication=Matrix(*)
  Reaching Rate : Constant  Value=20
  Sum : Sum  Inputs=|+-
  Sum3 : Sum  Inputs=|+-
  Transpose : Math  Operator=transpose
  phi : Constant  Value=0.0274
  x.dot.ref.ZERO : Ground
  u : Outport
  Slope : Outport  Port=2
  wires:
  Transpose/1 -> [C]
  [C] -> Product/1
  x/1 -> Sum3/2
  x_ref/1 -> Sum3/1
  Sum3/1 -> Product/2
  x.dot.ref.ZERO/1 -> Passthrough/1(In1)
  Passthrough/1(Out1) -> Sum/1
  f(x)/1 -> Sum/2
  Sum/1 -> Matrix Multiply/2
  [C] -> Matrix Multiply/1
  Product/1 -> Slope/1, Exponential Reaching/2(s), Boundary - Tangent/1(s(x))
  Control Gain/1 -> Exponential Reaching/4(K)
  Boundary - Tangent/1(z(s)) -> Exponential Reaching/1(z(s))
  Exponential Reaching/1(Out1) -> Add/1
  Matrix Multiply/1 -> Add/2
  [C] -> Product1/1
  g(x)/1 -> Product1/2
  Add/1 -> Divide/2
  Product1/1 -> Divide/1
  Divide/1 -> u/1
  Sliding Matrix/1 -> Transpose/1
  Phi/1 -> Boundary - Tangent/2(phi)
  Eta/1 -> Exponential Reaching/3(eta)

== system LQRconlacnguoc/Manual SMC Adaptive/Passthrough ==
  note: 1) Add Subsystem or Model blocks as valid variant choices.
      | 2) You cannot connect blocks at this level. At simulation, connectivity is automatically
      | determined, based on the active variant and port name matching.
  In1 : Inport
  Subsystem : Subsystem  VariantControl=true
  Subsystem1 : Subsystem  VariantControl=false
  Out1 : Outport

== system LQRconlacnguoc/Manual SMC Adaptive/Stable but chattery ==
  x : Inport
  x_ref : Inport  Port=2
  s(x) : Inport  Port=3
  MATLAB Function : MATLAB Function  TreatAsAtomicUnit=on
  C : Outport
  eta : Outport  Port=2
  phi : Outport  Port=3
  wires:
  s(x)/1 -> MATLAB Function/1(s)
  MATLAB Function/1(eta) -> eta/1
  MATLAB Function/2(phi) -> phi/1
  MATLAB Function/3(C) -> C/1
  x/1 -> MATLAB Function/2(x)
  x_ref/1 -> MATLAB Function/3(x_ref)

== system LQRconlacnguoc/Manual SMC Adaptive/Subsystem ==
  x : Inport
  x_ref : Inport  Port=2
  s(x) : Inport  Port=3
  MATLAB Function : MATLAB Function  TreatAsAtomicUnit=on
  C : Outport
  eta : Outport  Port=2
  phi : Outport  Port=3
  wires:
  s(x)/1 -> MATLAB Function/1(s)
  MATLAB Function/1(eta) -> eta/1
  MATLAB Function/2(phi) -> phi/1
  MATLAB Function/3(C) -> C/1
  x/1 -> MATLAB Function/2(x)
  x_ref/1 -> MATLAB Function/3(x_ref)

== system LQRconlacnguoc/STW SMC/Boundary - Tangent ==
  s(x) : Inport
  phi : Inport  Port=2
  Divide : Product  Inputs=*/
  Reshape1 : Reshape  OutputDimensionality=Column vector (2-D)
  Reshape2 : Reshape  OutputDimensionality=Column vector (2-D)
  Tanh : Trigonometry  Operator=tanh
  z(s) : Outport
  wires:
  Reshape1/1 -> Divide/2
  Divide/1 -> Tanh/1
  phi/1 -> Reshape1/1
  Reshape2/1 -> Divide/1
  Tanh/1 -> z(s)/1
  s(x)/1 -> Reshape2/1

== system LQRconlacnguoc/STW SMC/Exponential Reaching ==
  z(s) : Inport
  s : Inport  Port=2
  eta : Inport  Port=3
  K : Inport  Port=4
  Product : Product  Inputs=**
  Product1 : Product
  Sum : Sum  Inputs=--
  Out1 : Outport
  wires:
  z(s)/1 -> Product/2
  eta/1 -> Product/1
  s/1 -> Product1/1
  K/1 -> Product1/2
  Product/1 -> Sum/1
  Product1/1 -> Sum/2
  Sum/1 -> Out1/1

== system LQRconlacnguoc/STW SMC/Passthrough ==
  note: 1) Add Subsystem or Model blocks as valid variant choices.
      | 2) You cannot connect blocks at this level. At simulation, connectivity is automatically
      | determined, based on the active variant and port name matching.
  In1 : Inport
  Subsystem : Subsystem  VariantControl=true
  Subsystem1 : Subsystem  VariantControl=false
  Out1 : Outport

== system LQRconlacnguoc/Manual SMC/Passthrough/Subsystem ==
  In1 : Inport
  Out1 : Outport
  wires:
  In1/1 -> Out1/1

== system LQRconlacnguoc/Manual SMC/Passthrough/Subsystem1 ==
  In1 : Inport
  Out1 : Outport

== system LQRconlacnguoc/Manual SMC Adaptive/Manual SMC/Boundary - Tangent ==
  s(x) : Inport
  phi : Inport  Port=2
  Divide : Product  Inputs=*/
  Reshape1 : Reshape  OutputDimensionality=Column vector (2-D)
  Reshape2 : Reshape  OutputDimensionality=Column vector (2-D)
  Tanh : Trigonometry  Operator=tanh
  z(s) : Outport
  wires:
  Reshape1/1 -> Divide/2
  Divide/1 -> Tanh/1
  phi/1 -> Reshape1/1
  Reshape2/1 -> Divide/1
  Tanh/1 -> z(s)/1
  s(x)/1 -> Reshape2/1

== system LQRconlacnguoc/Manual SMC Adaptive/Manual SMC/Exponential Reaching ==
  z(s) : Inport
  s : Inport  Port=2
  eta : Inport  Port=3
  K : Inport  Port=4
  Product : Product  Inputs=**
  Product1 : Product
  Sum : Sum  Inputs=--
  Out1 : Outport
  wires:
  z(s)/1 -> Product/2
  eta/1 -> Product/1
  s/1 -> Product1/1
  K/1 -> Product1/2
  Product/1 -> Sum/1
  Product1/1 -> Sum/2
  Sum/1 -> Out1/1

== system LQRconlacnguoc/Manual SMC Adaptive/Manual SMC/Passthrough ==
  note: 1) Add Subsystem or Model blocks as valid variant choices.
      | 2) You cannot connect blocks at this level. At simulation, connectivity is automatically
      | determined, based on the active variant and port name matching.
  In1 : Inport
  Subsystem : Subsystem  VariantControl=true
  Subsystem1 : Subsystem  VariantControl=false
  Out1 : Outport

== system LQRconlacnguoc/Manual SMC Adaptive/Passthrough/Subsystem ==
  In1 : Inport
  Out1 : Outport
  wires:
  In1/1 -> Out1/1

== system LQRconlacnguoc/Manual SMC Adaptive/Passthrough/Subsystem1 ==
  In1 : Inport
  Out1 : Outport

== system LQRconlacnguoc/STW SMC/Passthrough/Subsystem ==
  In1 : Inport
  Out1 : Outport
  wires:
  In1/1 -> Out1/1

== system LQRconlacnguoc/STW SMC/Passthrough/Subsystem1 ==
  In1 : Inport
  Out1 : Outport

== system LQRconlacnguoc/Manual SMC Adaptive/Manual SMC/Passthrough/Subsystem ==
  In1 : Inport
  Out1 : Outport
  wires:
  In1/1 -> Out1/1

== system LQRconlacnguoc/Manual SMC Adaptive/Manual SMC/Passthrough/Subsystem1 ==
  In1 : Inport
  Out1 : Outport

== matlab function LQRconlacnguoc/Subsystem/MATLAB Function1 ==
  settings: updateMethod=DISCRETE
  data: x1 input; Kd_out output; x2 input; v1 input; v2 input; x2_ref input
function Kd_out = adaptive_Kd(x1, x2, v1, v2, x2_ref)
    persistent Kd_current e_prev;
    
    baseline_Kd = 5000;
    
    if isempty(Kd_current)
        Kd_current = baseline_Kd; 
        e_prev = [0; 0; 0; 0];
    end
    
    ref_x1 = 0; 
    ref_x2 = x2_ref; 
    ref_v1 = 0; 
    ref_v2 = 0;
    
    e = [(ref_x1 - x1); (ref_x2 - x2); (ref_v1 - v1); (ref_v2 - v2)];
         
    dt = 0.01; 
    
    e_dot = (e - e_prev) / dt;
    e_prev = e;
    
    rate_metric = abs(e' * e_dot); 
    
    % DRASTICALLY LOWER ALPHA
    alpha_3 = 2.8e4; % 400,000 instead of 40,000,000,000
    
    % NEW: THE LEAKAGE FACTOR (Sigma-Modification)
    sigma = 5; 
    
    % THE GRADIENT UPDATE RULE WITH LEAKAGE
    delta_Kd = (alpha_3 * rate_metric) - (sigma * (Kd_current - baseline_Kd));
    
    Kd_current = Kd_current + (delta_Kd * dt);
    
    max_Kd = 5500; 
    min_Kd = 3500; 
    
    if Kd_current > max_Kd
        Kd_current = max_Kd;
    elseif Kd_current < min_Kd
        Kd_current = min_Kd;
    end
    
    Kd_out = Kd_current;
end

== matlab function LQRconlacnguoc/Subsystem/MATLAB Function ==
  settings: updateMethod=DISCRETE
  data: x1 input; Kp_out output; x2 input; v1 input; v2 input; x2_ref input
function Kp_out = adaptive_Kp(x1, x2, v1, v2, x2_ref)
    persistent Kp_current;
    
    baseline_Kp = 10000; % Define baseline explicitly
    
    if isempty(Kp_current)
        Kp_current = baseline_Kp; 
    end
    
    ref_x1 = 0; 
    ref_x2 = x2_ref; 
    ref_v1 = 0; 
    ref_v2 = 0;
    
    e = [(ref_x1 - x1); (ref_x2 - x2); (ref_v1 - v1); (ref_v2 - v2)];
    
    total_error_energy = e' * e; 
    
    % DRASTICALLY LOWER ALPHA
    % Now, a 0.1m error will gently push the gain up, not instantly max it.
    alpha_1 = 9e4; % 500,000 instead of 50,000,000,000
    
    dt = 0.01; 
    
    % NEW: THE LEAKAGE FACTOR (Sigma-Modification)
    % This pulls the gain back to 12000 when the error is 0.
    sigma = 10; 
    
    % THE GRADIENT UPDATE RULE WITH LEAKAGE
    % If error is high, alpha wins. If error is low, sigma wins.
    delta_Kp = (alpha_1 * total_error_energy) - (sigma * (Kp_current - baseline_Kp));
    
    Kp_current = Kp_current + (delta_Kp * dt);
    
    max_Kp = 12000;
    min_Kp = 10000; 
    
    if Kp_current > max_Kp
        Kp_current = max_Kp;
    elseif Kp_current < min_Kp
        Kp_current = min_Kp;
    end
    
    Kp_out = Kp_current;
end

== matlab function LQRconlacnguoc/Manual SMC/Subsystem/MATLAB Function ==
  settings: updateMethod=DISCRETE  sampleTime=0.01
  data: s input; eta output; x input; x_ref input; phi output; C output
function [eta, phi, C] = culture_bees_smc(s, x, x_ref)
% Culture-Bees adaptive parameter optimizer for SMC
% Runs every sample, outputs updated eta, phi, C
% Parameters: (eta=η, phi=φ, C=sliding matrix)

%% ── PERSISTENT STATE (survives between time steps) ──────────────────
persistent belief_lambda belief_alpha belief_mu   % Belief space elites
persistent norm_lambda   norm_alpha   norm_mu     % Normative bounds
persistent initialized

%% ── ALGORITHM HYPERPARAMETERS (fixed, not adapted) ──────────────────
n_scout     = 10;   % number of Scout-Bees
n_selected  = 4;    % Selected-Bees (best sites)
n_recruit   = 20;   % Recruit-Bees per selected site
n_culture   = 4;    % Scout-Culture-Bees (40% of scout)
n_sel_cult  = 2;    % Selected-Culture-Bees (50% of culture)
N_belief    = 5;    % Belief space iterations

% Parameter bounds — enforce stability conditions
lambda_min = 0.5;  lambda_max = 15.0;
alpha_min  = 0.5;  alpha_max  = 25.0;
mu_min     = 0.01; mu_max     = 15.0;

% Patch sizes for neighbourhood search (Bees)
patch_alpha  = 0.0125;
patch_lambda = 0.0135;
patch_mu     = 0.0175;

% Patch sizes for belief space search (Cultural)
patch_c_alpha  = 0.01;
patch_c_lambda = 0.01;
patch_c_mu     = 0.01;

%% ── INITIALIZATION (first call only) ────────────────────────────────
if isempty(initialized)
    % Start belief space at reasonable centre values
    belief_lambda = 5.0;
    belief_alpha  = 10.0;
    belief_mu     = 1.0;

    % Normative knowledge — start with full bounds
    norm_lambda = [lambda_min, lambda_max];
    norm_alpha  = [alpha_min,  alpha_max];
    norm_mu     = [mu_min,     mu_max];

    initialized = true;
end

%% ── PART 1: BREEDING ENGINE ──────────────────────────────────────────
% Generate n_scout random candidate triplets within bounds
scouts = zeros(n_scout, 3);
for i = 1:n_scout
    scouts(i,1) = norm_lambda(1) + rand()*(norm_lambda(2)-norm_lambda(1)); % lambda
    scouts(i,2) = norm_alpha(1)  + rand()*(norm_alpha(2) -norm_alpha(1));  % alpha
    scouts(i,3) = norm_mu(1)     + rand()*(norm_mu(2)    -norm_mu(1));     % mu
end

%% ── PART 2: SEARCH ENGINE (Bees Algorithm) ───────────────────────────

% Evaluate all scouts
scout_mse = zeros(n_scout, 1);
for i = 1:n_scout
    scout_mse(i) = evaluate_mse(scouts(i,1), scouts(i,2), scouts(i,3), ...
                                 s, x, x_ref);
end

% Rank scouts — lower MSE = better
[~, idx] = sort(scout_mse, 'ascend');
selected = scouts(idx(1:n_selected), :);

% Neighbourhood search around each selected site
best_recruit    = zeros(n_selected, 3);
best_recruit_mse = zeros(n_selected, 1);

for i = 1:n_selected
    site = selected(i, :);
    recruits     = zeros(n_recruit, 3);
    recruit_mse  = zeros(n_recruit, 1);

    for j = 1:n_recruit
        % Perturb around site using patch sizes
        d_lambda = patch_lambda * site(1) * (rand() - 0.5);
        d_alpha  = patch_alpha  * site(2) * (rand() - 0.5);
        d_mu     = patch_mu     * site(3) * (rand() - 0.5);

        candidate = [site(1)+d_lambda, site(2)+d_alpha, site(3)+d_mu];

        % Enforce bounds
        candidate(1) = clamp(candidate(1), lambda_min, lambda_max);
        candidate(2) = clamp(candidate(2), alpha_min,  alpha_max);
        candidate(3) = clamp(candidate(3), mu_min,     mu_max);

        recruits(j,:)    = candidate;
        recruit_mse(j)   = evaluate_mse(candidate(1), candidate(2), ...
                                         candidate(3), s, x, x_ref);
    end

    % Pick fittest recruit
    [best_recruit_mse(i), best_j] = min(recruit_mse);
    best_recruit(i,:) = recruits(best_j,:);
end

% Fittest-Bees: best recruit from each selected site
[~, fittest_idx] = sort(best_recruit_mse, 'ascend');
fittest_bees     = best_recruit(fittest_idx, :);
fittest_mse      = best_recruit_mse(fittest_idx);

%% ── PART 3: AGGREGATION KNOWLEDGE ENGINE (Cultural Algorithm) ────────

% Take top 40% of fittest bees as Scout-Culture-Bees
n_sc = max(1, round(0.4 * n_selected));
scout_culture     = fittest_bees(1:n_sc, :);
scout_culture_mse = fittest_mse(1:n_sc);

% Acceptance: select top 50% as Selected-Culture-Bees
n_scc = max(1, round(0.5 * n_sc));
[~, sc_idx]    = sort(scout_culture_mse, 'ascend');
sel_culture    = scout_culture(sc_idx(1:n_scc), :);

% Update situational knowledge (best elite seen)
best_sc_mse = scout_culture_mse(sc_idx(1));
current_belief_mse = evaluate_mse(belief_lambda, belief_alpha, belief_mu, ...
                                   s, x, x_ref);
if best_sc_mse < current_belief_mse
    belief_lambda = sel_culture(1,1);
    belief_alpha  = sel_culture(1,2);
    belief_mu     = sel_culture(1,3);
end

% Belief space search loop
best_belief_lambda = belief_lambda;
best_belief_alpha  = belief_alpha;
best_belief_mu     = belief_mu;
best_belief_mse    = current_belief_mse;

for iter = 1:N_belief
    % Generate Recruit-Culture-Bees around belief
    d_lc = patch_c_lambda * belief_lambda * (rand() - 0.5);
    d_ac = patch_c_alpha  * belief_alpha  * (rand() - 0.5);
    d_mc = patch_c_mu     * belief_mu     * (rand() - 0.5);

    cand_l = clamp(belief_lambda + d_lc, lambda_min, lambda_max);
    cand_a = clamp(belief_alpha  + d_ac, alpha_min,  alpha_max);
    cand_m = clamp(belief_mu     + d_mc, mu_min,     mu_max);

    cand_mse = evaluate_mse(cand_l, cand_a, cand_m, s, x, x_ref);

    % Accept if better AND within normative bounds
    in_norm = (cand_l >= norm_lambda(1)) && (cand_l <= norm_lambda(2)) && ...
              (cand_a >= norm_alpha(1))  && (cand_a <= norm_alpha(2))  && ...
              (cand_m >= norm_mu(1))     && (cand_m <= norm_mu(2));

    if cand_mse < best_belief_mse && in_norm
        best_belief_lambda = cand_l;
        best_belief_alpha  = cand_a;
        best_belief_mu     = cand_m;
        best_belief_mse    = cand_mse;
    end
end

% Update normative knowledge bounds toward successful region
norm_lambda = update_norm(norm_lambda, best_belief_lambda, lambda_min, lambda_max);
norm_alpha  = update_norm(norm_alpha,  best_belief_alpha,  alpha_min,  alpha_max);
norm_mu     = update_norm(norm_mu,     best_belief_mu,     mu_min,     mu_max);

% Final adaptive outputs
belief_lambda = best_belief_lambda;
belief_alpha  = best_belief_alpha;
belief_mu     = best_belief_mu;

%% ── MAP TO SMC BLOCK PARAMETERS ─────────────────────────────────────
eta  = belief_alpha;                        % η  ← α
phi  = 1 / belief_mu;                       % φ  ← 1/μ (Simulink uses tanh(s/φ))
C    = belief_lambda * [0; 1; 0; 1];        % C  ← λ scales [c2, c4] weights
                                             % adjust shape vector to your plant

end % main function

%% ══════════════════════════════════════════════════════════════════════
%% LOCAL FUNCTION: MSE COST EVALUATOR
%% ══════════════════════════════════════════════════════════════════════
function mse = evaluate_mse(lambda, alpha, mu, s, x, x_ref)
% Compute the cost of a given (lambda, alpha, mu) triplet
% given the current system state
%
% We cannot simulate forward in this optimizer (no plant model here),
% so we use a PROXY cost based on current sliding surface behavior:
%
%   Cost = position tracking error² + velocity tracking error²
%          + chattering penalty (large alpha with small s = wasteful)
%          + surface penalty (|s| should be small)

    e_pos = (x_ref(3) - x(3))^2;          % x2 position error squared
    e_vel = (x_ref(4) - x(4))^2;          % x2 velocity error squared

    % Surface magnitude penalty
    s_penalty = s^2;

    % Chattering penalty: large alpha when near surface is wasteful
    chat_penalty = (alpha / (mu + 0.001)) * exp(-abs(s));

    % Equivalent control effort proxy:
    % large lambda with large error = good (fast convergence)
    % large lambda with small error = bad (overshoot risk)
    lambda_penalty = lambda^2 * exp(-abs(s)) * (e_pos + e_vel);

    mse = e_pos + e_vel + 0.1*s_penalty + 0.05*chat_penalty + 0.1*lambda_penalty;
end

%% ══════════════════════════════════════════════════════════════════════
%% LOCAL FUNCTION: CLAMP
%% ══════════════════════════════════════════════════════════════════════
function val = clamp(val, lo, hi)
    if val < lo; val = lo; end
    if val > hi; val = hi; end
end

%% ══════════════════════════════════════════════════════════════════════
%% LOCAL FUNCTION: NORMATIVE KNOWLEDGE UPDATER
%% ══════════════════════════════════════════════════════════════════════
function bounds = update_norm(bounds, best_val, hard_min, hard_max)
% Shrink normative bounds toward the successful region
% but never violate the hard stability bounds
    shrink = 0.05;  % how fast bounds tighten (5% per step)
    range  = bounds(2) - bounds(1);

    new_lo = max(hard_min, bounds(1) + shrink * (best_val - bounds(1)));
    new_hi = min(hard_max, bounds(2) - shrink * (bounds(2) - best_val));

    % Never let bounds collapse too tightly
    if (new_hi - new_lo) < 0.1 * range
        new_lo = max(hard_min, best_val - 0.05*range);
        new_hi = min(hard_max, best_val + 0.05*range);
    end

    bounds = [new_lo, new_hi];
end
